simulink subsystem "Vision_Relative_Errors_sub"  (R2023b)
settings: Solver=VariableStepAuto  StartTime=0.0  StopTime=10.0  RelTol=1e-3
undefined symbols (not defined in the file): Relative_Steering_Error_Angle_Gain_Object_Factor, TEST_Pipeline, Vision_Object_Target_Angle, Vision_Object_Target_X, Vision_Object_Target_Y, Vision_Tag_Target_Angle, Vision_Tag_Target_X, Vision_Tag_Target_Y
libraries: simulink x6
settings Model: Creator=ander  LastModifiedBy=ander

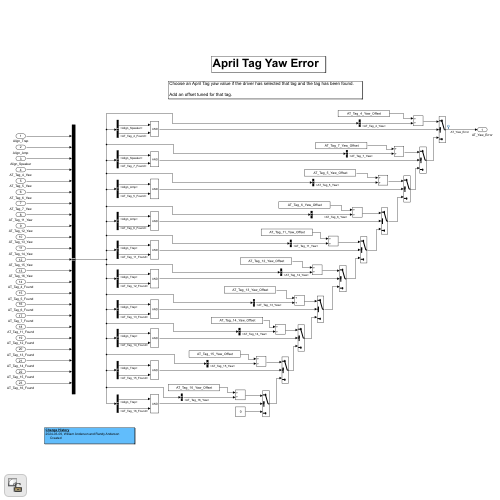
[thumbnail: Simulink's stored preview of the top-level diagram]
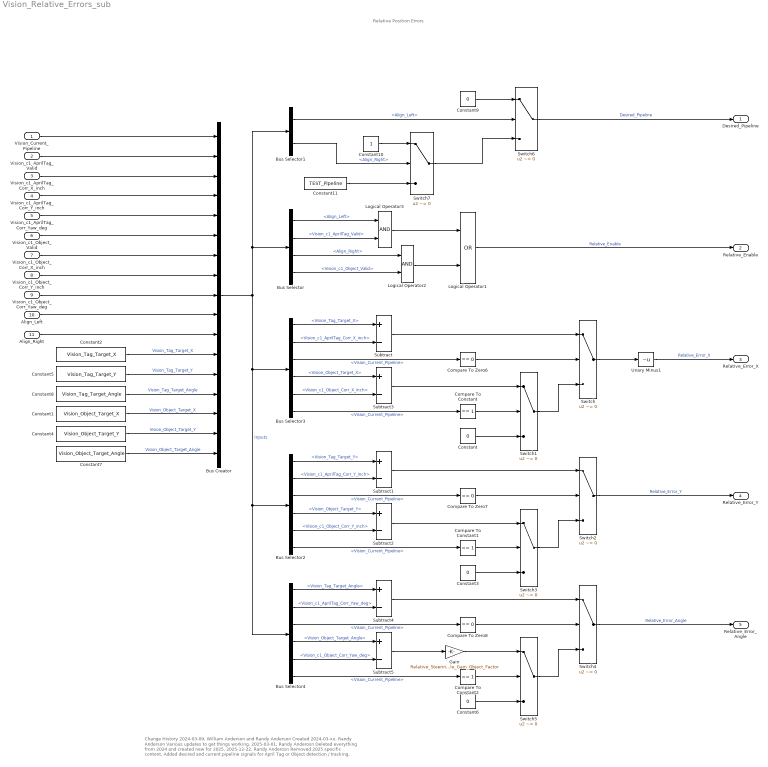
== system Vision_Relative_Errors_sub ==
  note: Change History
      | 2024-03-09, William Anderson and Randy Anderson
      | Created
      | 2024-03-xx, Randy Anderson
      | Various updates to get things working.
      | 2025-03-01, Randy Anderosn
      | Deleted everything from 2024 and created new for 2025.
      | 2025-12-22, Randy Anderosn
      | Removed 2025 specific content.
      | Added desired and current pipeline signals for April Tag or Object detection / tracking.
  note: Relative Position Errors
  Vision_Current_Pipeline : Inport
  Vision_c1_AprilTag_Valid : Inport  Port=2
  Vision_c1_AprilTag_Corr_X_inch : Inport  Port=3
  Vision_c1_AprilTag_Corr_Y_inch : Inport  Port=4
  Vision_c1_AprilTag_Corr_Yaw_deg : Inport  Port=5
  Vision_c1_Object_Valid : Inport  Port=6
  Vision_c1_Object_Corr_X_inch : Inport  Port=7
  Vision_c1_Object_Corr_Y_inch : Inport  Port=8
  Vision_c1_Object_Corr_Yaw_deg : Inport  Port=9
  Align_Left : Inport  Port=10
  Align_Right : Inport  Port=11
  Bus Creator : BusCreator  Inputs=17
  Bus Selector : BusSelector  OutputSignals=Align_Left,Vision_c1_AprilTag_Valid,Align_Right,Vision_c1_Object_Valid
  Bus Selector1 : BusSelector  OutputSignals=Align_Left,Align_Right
  Bus Selector2 : BusSelector  OutputSignals=Vision_Tag_Target_Y,Vision_c1_AprilTag_Corr_Y_inch,Vision_Current_Pipeline,Vision_Object_Target_Y,Vision_c1_Object_Corr_Y_inch,Vision_Current_Pipeline
  Bus Selector3 : BusSelector  OutputSignals=Vision_Tag_Target_X,Vision_c1_AprilTag_Corr_X_inch,Vision_Current_Pipeline,Vision_Object_Target_X,Vision_c1_Object_Corr_X_inch,Vision_Current_Pipeline
  Bus Selector4 : BusSelector  OutputSignals=Vision_Tag_Target_Angle,Vision_c1_AprilTag_Corr_Yaw_deg,Vision_Current_Pipeline,Vision_Object_Target_Angle,Vision_c1_Object_Corr_Yaw_deg,Vision_Current_Pipeline
  Compare To Constant : simulink/Logic and Bit Operations/Compare To Constant  relop===  const=1  OutDataTypeStr=boolean
  Compare To Constant1 : simulink/Logic and Bit Operations/Compare To Constant  relop===  const=1  OutDataTypeStr=boolean
  Compare To Constant2 : simulink/Logic and Bit Operations/Compare To Constant  relop===  const=1  OutDataTypeStr=boolean
  Compare To Zero6 : simulink/Logic and Bit Operations/Compare To Zero  relop===  OutDataTypeStr=boolean
  Compare To Zero7 : simulink/Logic and Bit Operations/Compare To Zero  relop===  OutDataTypeStr=boolean
  Compare To Zero8 : simulink/Logic and Bit Operations/Compare To Zero  relop===  OutDataTypeStr=boolean
  Constant : Constant  Value=0
  Constant1 : Constant  Value=Vision_Object_Target_X
  Constant10 : Constant  OutDataTypeStr=uint8
  Constant11 : Constant  Value=TEST_Pipeline
  Constant2 : Constant  Value=Vision_Tag_Target_X
  Constant3 : Constant  Value=0
  Constant4 : Constant  Value=Vision_Object_Target_Y
  Constant5 : Constant  Value=Vision_Tag_Target_Y
  Constant6 : Constant  Value=0
  Constant7 : Constant  Value=Vision_Object_Target_Angle
  Constant8 : Constant  Value=Vision_Tag_Target_Angle
  Constant9 : Constant  Value=0  OutDataTypeStr=uint8
  Gain : Gain  Gain=Relative_Steering_Error_Angle_Gain_Object_Factor
      settings: AttributesFormatString=%<Gain>
  Logical Operator1 : Logic  Operator=OR  AllPortsSameDT=off  OutDataTypeStr=boolean
  Logical Operator2 : Logic  AllPortsSameDT=off  OutDataTypeStr=boolean
  Logical Operator3 : Logic  AllPortsSameDT=off  OutDataTypeStr=boolean
  Subtract{,1..5} (6 alike) : Sum  Inputs=+-
  Switch{,1..7} (8 alike) : Switch  Criteria=u2 ~= 0  SaturateOnIntegerOverflow=off  InputSameDT=off
  Unary Minus1 : UnaryMinus
  Desired_Pipeline : Outport
  Relative_Enable : Outport  Port=2
  Relative_Error_X : Outport  Port=3
  Relative_Error_Y : Outport  Port=4
  Relative_Error_Angle : Outport  Port=5
  wires:
  Bus Creator/1 -> Bus Selector3/1, Bus Selector4/1, Bus Selector2/1, Bus Selector1/1, Bus Selector/1  "Inputs"
  Logical Operator1/1 -> Relative_Enable/1  "Relative_Enable"
  Switch2/1 -> Relative_Error_Y/1  "Relative_Error_Y"
  Switch4/1 -> Relative_Error_Angle/1  "Relative_Error_Angle"
  Unary Minus1/1 -> Relative_Error_X/1  "Relative_Error_X"
  Switch1/1 -> Switch/3
  Constant/1 -> Switch1/3
  Bus Selector1/1 -> Switch6/2  "<Align_Left>"
  Bus Selector1/2 -> Switch7/2  "<Align_Right>"
  Switch7/1 -> Switch6/3
  Switch6/1 -> Desired_Pipeline/1  "Desired_Pipeline"
  Constant9/1 -> Switch6/1
  Constant10/1 -> Switch7/1
  Constant11/1 -> Switch7/3
  Subtract/1 -> Switch/1
  Subtract3/1 -> Switch1/1
  Switch/1 -> Unary Minus1/1
  Align_Right/1 -> Bus Creator/11
  Align_Left/1 -> Bus Creator/10
  Vision_Current_Pipeline/1 -> Bus Creator/1
  Vision_c1_AprilTag_Corr_X_inch/1 -> Bus Creator/3
  Vision_c1_AprilTag_Corr_Y_inch/1 -> Bus Creator/4
  Vision_c1_AprilTag_Corr_Yaw_deg/1 -> Bus Creator/5
  Compare To Zero6/1 -> Switch/2
  Bus Selector3/2 -> Subtract/2  "<Vision_c1_AprilTag_Corr_X_inch>"
  Compare To Constant/1 -> Switch1/2
  Compare To Zero7/1 -> Switch2/2
  Subtract2/1 -> Switch3/1
  Subtract1/1 -> Switch2/1
  Switch3/1 -> Switch2/3
  Constant3/1 -> Switch3/3
  Compare To Constant1/1 -> Switch3/2
  Constant6/1 -> Switch5/3
  Subtract4/1 -> Switch4/1
  Switch5/1 -> Switch4/3
  Compare To Constant2/1 -> Switch5/2
  Compare To Zero8/1 -> Switch4/2
  Bus Selector/1 -> Logical Operator3/1  "<Align_Left>"
  Constant2/1 -> Bus Creator/12  "Vision_Tag_Target_X"
  Constant5/1 -> Bus Creator/13  "Vision_Tag_Target_Y"
  Constant8/1 -> Bus Creator/14  "Vision_Tag_Target_Angle"
  Constant1/1 -> Bus Creator/15  "Vision_Object_Target_X"
  Constant4/1 -> Bus Creator/16  "Vision_Object_Target_Y"
  Constant7/1 -> Bus Creator/17  "Vision_Object_Target_Angle"
  Bus Selector3/1 -> Subtract/1  "<Vision_Tag_Target_X>"
  Bus Selector3/3 -> Compare To Zero6/1  "<Vision_Current_Pipeline>"
  Bus Selector3/4 -> Subtract3/1  "<Vision_Object_Target_X>"
  Bus Selector3/5 -> Subtract3/2  "<Vision_c1_Object_Corr_X_inch>"
  Bus Selector3/6 -> Compare To Constant/1  "<Vision_Current_Pipeline>"
  Bus Selector2/1 -> Subtract1/1  "<Vision_Tag_Target_Y>"
  Bus Selector2/2 -> Subtract1/2  "<Vision_c1_AprilTag_Corr_Y_inch>"
  Bus Selector2/3 -> Compare To Zero7/1  "<Vision_Current_Pipeline>"
  Bus Selector2/4 -> Subtract2/1  "<Vision_Object_Target_Y>"
  Bus Selector2/5 -> Subtract2/2  "<Vision_c1_Object_Corr_Y_inch>"
  Bus Selector2/6 -> Compare To Constant1/1  "<Vision_Current_Pipeline>"
  Bus Selector4/1 -> Subtract4/1  "<Vision_Tag_Target_Angle>"
  Bus Selector4/2 -> Subtract4/2  "<Vision_c1_AprilTag_Corr_Yaw_deg>"
  Bus Selector4/3 -> Compare To Zero8/1  "<Vision_Current_Pipeline>"
  Bus Selector4/4 -> Subtract5/1  "<Vision_Object_Target_Angle>"
  Bus Selector4/5 -> Subtract5/2  "<Vision_c1_Object_Corr_Yaw_deg>"
  Bus Selector4/6 -> Compare To Constant2/1  "<Vision_Current_Pipeline>"
  Vision_c1_Object_Corr_X_inch/1 -> Bus Creator/7
  Vision_c1_Object_Corr_Y_inch/1 -> Bus Creator/8
  Vision_c1_Object_Corr_Yaw_deg/1 -> Bus Creator/9
  Logical Operator3/1 -> Logical Operator1/1
  Subtract5/1 -> Gain/1
  Gain/1 -> Switch5/1
  Vision_c1_AprilTag_Valid/1 -> Bus Creator/2
  Vision_c1_Object_Valid/1 -> Bus Creator/6
  Bus Selector/2 -> Logical Operator3/2  "<Vision_c1_AprilTag_Valid>"
  Bus Selector/3 -> Logical Operator2/1  "<Align_Right>"
  Bus Selector/4 -> Logical Operator2/2  "<Vision_c1_Object_Valid>"
  Logical Operator2/1 -> Logical Operator1/2
